simulink model "TB23_R2_SALS_Link"  (R2025a)
settings: Solver=FixedStepDiscrete  StartTime=0  StopTime=TB.t_end  FixedStep=TB.dt  RelTol=1e-3
InitFcn:
  | % 모델과 같은 폴더의 초기화 스크립트를 실행해 P(설계 파라미터)와 TB(시험 조건)를 만든다.
  | run(fullfile(fileparts(get_param(bdroot, 'FileName')), 'TB23_init.m'));
values from neighbouring files (symbols this model uses):
  TB = struct()    [TB23_init.m]    (also in run_TB23.m = evalin('base', 'TB'))
libraries: fl_lib x71, nesl_utility x31
(part 3 of 3)

== matlab function TB23_R2_SALS_Link/Gate_StageB/StageB_Gate ==
  data: t input; g output; uc input; ilink input; prm input; init input; eps input; aux output
function [g, aux] = prism_gate_stageB_f(t, uc, ilink, prm, init, eps)
%#codegen
%PRISM_GATE_STAGEB_F  Stage B 게이트 생성기 + DAB 고장 모드 변조(EPS) + 직류 편류 없는 지령 전이(TB12).
%
%  ctrl/prism_gate_stageB_e.m(TB10·TB11)과 같고, EPS 지령이 바뀔 때의 전이만 다르다(TB11에서 지령표 칸 전환으로
%  (D1, φ)가 한 번에 0.1·0.23 rad 바뀐 주기에 누설 전류에 직류 편류가 생겨 첨두가 88.5 A까지 올랐다).
%    1) 레그 2 지연(D1)이 바뀌면 그 뒤 첫 레그 2 에지는 이전·새 값의 중간(반 이동), 다음 에지부터 새 값을 쓴다.
%       구형파 레그 하나의 에지가 Δ 옮겨질 때 첫 에지를 Δ/2만 옮기면 그 레그가 만드는 인덕터 전류에 직류 편류가 남지 않는다
%       (SPS 위상의 전이 반주기 평균과 같은 원리를 레그마다 적용). 이전 판(e)은 D1을 한 주기 동안 그대로 잡았다.
%    2) EPS 위상은 반주기마다 SPH = 0.01 rad, D1은 에지마다 SD1 = 0.005까지만 옮긴다(지령표의 큰 칸 전환을 수 주기에 나눔).
%       EPS가 켜질 때는 지금 쓰던 SPS 위상에서 출발한다. 정상 붕괴 중의 지령 변화(주기당 D1 약 0.0006)보다 훨씬 크므로
%       평소 동작에는 영향이 없다.
%  EPS가 꺼져 있으면(eps(1) = 0) prism_gate_stageB.m·prism_gate_stageB_e.m과 같은 게이트를 낸다.
%  아래는 이전 판 설명:
%PRISM_GATE_STAGEB_E(이전 판)  Stage B 게이트 생성기 + DAB 고장 모드 변조(EPS, TB10). eps(1) = 0이면 ctrl/prism_gate_stageB.m과 같다.
%
%  EPS(1차 내부 위상천이): SPS 생성기가 정한 1차 에지(가상 에지)에서 레그 1(P1·P2)은 그대로 바꾸고, 레그 2(P3·P4)는
%  D1·T/2 늦게 바꾼다. 1차 전압은 −V → 0(레그 1만 바뀜) → +V(레그 2도 바뀜)가 되어 반주기마다 (1 − D1)·T/2 폭의 펄스가 된다.
%  D1은 상향 가상 에지에서 잡아 그 주기의 하향 에지까지 그대로 쓴다(양·음 펄스 폭이 같아 1차 직류 편류가 생기지 않는다).
%  위상은 eps(2)를 SPS 위상 지령 대신 쓰므로, 위상 변화의 직류 편류 방지(전이 반주기 평균)는 SPS와 같이 적용된다.
%  위상 기준: 2차 상향 에지 − 가상 에지 = φ, 1차 펄스 시작 = 가상 에지 + D1·T/2(검증 코드 dab_modulation.eps_params와 같은 정의).
%
%  추가 입력  eps  [EPS 켬(1/0); 위상 φ [rad]; 내부 위상비 D1(0–0.95)]  (ctrl/prism_dab_eps_map.m)
%
%  아래는 SPS 생성기 설명(그대로):
%PRISM_GATE_STAGEB  Stage B 게이트 생성기(적분 간격 dt = 5 ns마다 실행).
%
%  H-브리지 : 유니폴라 PWM. 삼각 반송파 c(t)는 제어주기 시작(표본 시점)에서 +1, 반주기에서 −1.
%             레그 A 상측 목표 = (m > c), 레그 B 상측 목표 = (−m > c). 목표가 바뀌면 두 소자를 데드타임 동안
%             끄고(출력용량 충방전·다이오드 도통은 회로가 정함) 새 소자를 켠다.
%  DAB      : 50 % 구형파 두 풀브리지, 단일 위상천이. 에지는 반송파 반주기 중심 c_j에 대칭(1차 c_j − δ/2,
%             2차 c_j + δ/2, δ = φ·T/2π)으로 놓고, 지령은 도착 후 첫 반주기 중심에서 반영한다.
%             전이 반주기의 위상차를 이전·새 위상의 평균으로 두는 갱신(A ← −A + 2Δ, Δ = (A + δ_new)/2)으로
%             위상이 바뀔 때 변압기 직류 편류가 생기지 않게 한다(검증 코드와 같은 알고리즘).
%             에지 시각은 dt 격자에 반올림하고, 실제 실행 시각으로 다음 반주기의 A를 계산한다.
%  링크전류 : DAB 2차 브리지가 링크로 보내는 직류전류를 제어주기마다 평균해 다음 표본에 넘긴다.
%
%  입력  t      시뮬레이션 시각(Digital Clock, dt 간격)
%        uc     [PWM 비교값; DAB 유효 위상 rad]  (제어기 출력, 전달지연 뒤)
%        ilink  DAB 2차 브리지 → 링크 직류전류 [A](순시)
%        prm    [dt Np td_h(간격 수) td_d(간격 수) T]
%        init   [PWM 비교값 초기값, 위상 초기값, 링크전류 초기값]
%  출력  g      [A상측 A하측 B상측 B하측 | P1 P2 P3 P4 | S1 S2 S3 S4]  (1 = 켬)
%               DAB 브리지: 상태 +1 → 1·4번 켬, −1 → 2·3번 켬(1·2번이 레그 1, 3·4번이 레그 2, 홀수 = 상측)
%        aux    [링크전류 주기 평균; 그 주기 두 반주기 중심의 위상 φ_c0, φ_c1; 반송파; 1차 상태; 2차 상태]

persistent started kA kB tgtA tgtB A ph_tgt p_t s_t p_h s_h p_j s_j p_state s_state p_te s_te ...
           acc il_avg phc0 phc1 lat0 lat1 D1c l2_t l2_tgt l2_hi l2_te l2_pend D1p ph_e e_on
dt = prm(1); Np = prm(2); ndh = prm(3); ndd = prm(4); T = prm(5);
Nh = round(Np/2);
k  = round(t/dt);                     % 적분 간격 번호(0부터)
t0 = k*dt;

if isempty(started)
    started = 1;
    m0 = init(1); ph0 = init(2);
    c0 = 1;                            % k = 0의 반송파
    tgtA = double(m0 > c0); tgtB = double(-m0 > c0);
    kA = -1e9; kB = -1e9;              % 데드타임 없이 시작
    ph_tgt = ph0;
    d0 = ph0/(2*pi)*T;
    A = d0;
    p_t = [1e30 1e30]; s_t = [1e30 1e30]; p_h = [0 0]; s_h = [0 0];
    p_te = -1; s_te = -1;
    if d0 > 0
        p_j = 1; p_h(1) = -d0/2; p_state = 1;  s_j = 0; s_state = -1;
    elseif d0 < 0
        s_j = 1; s_h(1) = d0/2;  s_state = 1;  p_j = 0; p_state = -1;
    else
        p_j = 0; s_j = 0; p_state = -1; s_state = -1;
    end
    acc = 0; il_avg = init(3); phc0 = ph0; phc1 = ph0; lat0 = ph0; lat1 = ph0;
    D1c = 0; D1p = 0; ph_e = 0; e_on = 0; l2_t = 1e30; l2_tgt = double(p_state < 0); l2_hi = l2_tgt; l2_te = -1; l2_pend = 0;
end

m = uc(1);
SPH = 0.01;                           % EPS 위상 변화율 상한 [rad/반주기]
SD1 = 0.005;                          % EPS D1 변화율 상한 [/반주기]
if eps(1) > 0.5
    if ~e_on, ph_e = ph_tgt; e_on = 1; end           % 켜질 때 지금 쓰는 SPS 위상에서 출발
    if mod(k, Nh) == 0                               % 반주기 중심에서만 위상 지령을 한 단계 옮긴다
        dphi = mod(eps(2) - ph_e + pi, 2*pi) - pi;
        ph_e = ph_e + min(max(dphi, -SPH), SPH);
    end
    ph_tgt = ph_e;
else
    e_on = 0;
    ph_tgt = uc(2);
end

% ---------------- H-브리지 유니폴라 PWM -------------------------------------------------
kin = mod(k, Np);
c = 4*abs(kin/Np - 0.5) - 1;
nA = double(m > c); nB = double(-m > c);
if nA ~= tgtA, tgtA = nA; kA = k; end
if nB ~= tgtB, tgtB = nB; kB = k; end
okA = (k - kA) >= ndh; okB = (k - kB) >= ndh;
gA_hi = double(okA && tgtA == 1); gA_lo = double(okA && tgtA == 0);
gB_hi = double(okB && tgtB == 1); gB_lo = double(okB && tgtB == 0);

% ---------------- DAB 위상 갱신(반주기 중심) --------------------------------------------
if mod(k, Nh) == 0
    j = k/Nh; cj = t0;
    if j >= 1
        jm = mod(j - 1, 2) + 1;
        A = -A + 2*(s_h(jm) - p_h(jm));
    end
    dtg = ph_tgt/(2*pi)*T;
    D = 0.5*(A + dtg);
    jj = mod(j, 2) + 1;
    p_done = p_j > j; s_done = s_j > j;
    if p_done && ~s_done
        s_t(jj) = max(cj, p_h(jj) + D);
    elseif s_done && ~p_done
        p_t(jj) = max(cj, s_h(jj) - D);
    elseif ~p_done && ~s_done
        if D >= 0
            p_t(jj) = cj; s_t(jj) = cj + D;
        else
            s_t(jj) = cj; p_t(jj) = cj - D;
        end
    end
    if p_done, tpj = p_h(jj); else, tpj = p_t(jj); end
    if s_done, tsj = s_h(jj); else, tsj = s_t(jj); end
    D1 = 0.5*(-A + 2*(tsj - tpj) + dtg);
    cn = (j + 1)*Nh*dt;
    p_t(3 - jj) = cn - D1/2; s_t(3 - jj) = cn + D1/2;
    if mod(j, 2) == 0, phc0 = ph_tgt; else, phc1 = ph_tgt; end
end
% ---------------- DAB 에지 실행(가장 가까운 간격에 반올림) ------------------------------
sp = mod(p_j, 2) + 1;
if p_t(sp) < t0 + 0.5*dt
    if mod(p_j, 2) == 0, p_state = 1; else, p_state = -1; end
    if eps(1) > 0.5, D1n = min(max(eps(3), 0), 0.95); else, D1n = 0; end
    D1n = D1p + min(max(D1n - D1p, -SD1), SD1);      % 에지마다 D1 변화율 제한
    if abs(D1n - D1p) > 1e-9
        D1c = 0.5*(D1p + D1n);        % 레그 2 지연이 바뀌면 첫 에지는 중간값(반 이동), 다음 에지부터 새 값: 직류 편류 없음
        D1p = D1n;
    else
        D1c = D1n;
    end
    p_te = t0; p_h(sp) = t0; p_t(sp) = 1e30; p_j = p_j + 1;
    if l2_pend > 0.5                   % (위상 전이로 반주기가 짧아진 경우) 남은 레그 2 전환을 먼저 끝낸다
        l2_hi = l2_tgt; l2_te = t0; l2_pend = 0;
    end
    l2_tgt = double(p_state < 0); l2_t = t0 + D1c*T/2; l2_pend = 1;   % 레그 2: −1 상태에서 상측(P3) 켬
end
if l2_pend > 0.5 && l2_t < t0 + 0.5*dt
    l2_hi = l2_tgt; l2_te = t0; l2_pend = 0;
end
ss = mod(s_j, 2) + 1;
if s_t(ss) < t0 + 0.5*dt
    if mod(s_j, 2) == 0, s_state = 1; else, s_state = -1; end
    s_te = t0; s_h(ss) = t0; s_t(ss) = 1e30; s_j = s_j + 1;
end
p_ok = (t0 - p_te) >= ndd*dt - 0.5*dt;
s_ok = (t0 - s_te) >= ndd*dt - 0.5*dt;
gP = [0 0 0 0]; gS = [0 0 0 0];
if p_ok                                % 레그 1(P1 상측, P2 하측)
    if p_state > 0, gP(1:2) = [1 0]; else, gP(1:2) = [0 1]; end
end
if (t0 - l2_te) >= ndd*dt - 0.5*dt     % 레그 2(P3 상측, P4 하측), 자기 전환 뒤 데드타임
    if l2_hi > 0.5, gP(3:4) = [1 0]; else, gP(3:4) = [0 1]; end
end
if s_ok
    if s_state > 0, gS = [1 0 0 1]; else, gS = [0 1 1 0]; end
end

% ---------------- 링크전류 주기 평균(표본 직전 간격에서 확정) -------------------------
acc = acc + ilink;
if kin == Np - 1
    il_avg = acc/Np; acc = 0;
    lat0 = phc0; lat1 = phc1;
end

g = [gA_hi gA_lo gB_hi gB_lo gP gS]';
aux = [il_avg; lat0; lat1; c; p_state; s_state];
end

== matlab function TB23_R2_SALS_Link/Gate_StageB/R2_Gate_Protect ==
  data: t input; gb output; g input; sup input; meas input; prm input; fl output
function [gb, fl] = prism_r2_gate_b(t, g, sup, meas, prm)
%#codegen
%PRISM_R2_GATE_B  R2 보호 상태기계의 게이트 재정의(TB09, 적분 간격마다 실행): 하드웨어 비교기, 고장 주입, 모드별 게이트.
%
%  입력  g     게이트 생성기 출력 [A상측 A하측 B상측 B하측 | P1–P4 | S1–S4] (ctrl/prism_gate_stageB.m)
%        sup   상태기계 지령 [브리지 모드(0 제어 PWM, 1 영벡터, 2 차단, 3 조향 PWM); DAB 모드(0 제어기, 1 보조, 2 정지);
%              바이패스 주 스위치; 제동 저항 게이트; 상태 번호]
%        meas  [i_p i_h v_link v_s v_bus]
%        prm   [dt T_HW I_HW VL_HW VS_HW 상한 고장종류(0 없음, 1 H-브리지 개방, 2 DAB 정지) 고장시각 T_GDF (두 번째 고장 시각)]
%              (TB23) 10번째 값이 있으면 그 시각에 비교기 차단 래치를 강제로 켠다(DAB 고장 강등 중 H-브리지 차단 → 이중 고장)
%  출력  gb    [H-브리지 4 | DAB 8 | 바이패스 주 스위치 | 제동 저항]
%        fl    [게이트 구동기 고장 신호(H-브리지 개방, T_GDF 뒤); 하드웨어 비교기 차단 래치]
%  하드웨어 비교기는 H-브리지가 동작하는 동안(차단·고장 전) 연속 감시한다: |i_p|·|i_h| > I_HW, v_link > VL_HW,
%  |v_s| > VS_HW, 그리고 정상 조정 상태(1–5)에서 v_bus > 부품 등급 상한. 조건이 T_HW 동안 이어지면 브리지를 끄고 래치한다.

persistent since trip
if isempty(trip), since = -1; trip = 0; end
T_HW = prm(2); I_HW = prm(3); VL_HW = prm(4); VS_HW = prm(5); upper = prm(6);
ftype = prm(7); t_f = prm(8); T_GDF = prm(9);
bmode = round(sup(1)); dmode = round(sup(2)); st = round(sup(5));
hb_fault = ftype == 1 && t >= t_f;
dab_fault = ftype == 2 && t >= t_f;
ip = meas(1); ih = meas(2); vl = meas(3); vs = meas(4); vb = meas(5);
if trip < 0.5 && ~hb_fault && bmode ~= 2
    normal = st >= 1 && st <= 5;
    cond = abs(ip) > I_HW || abs(ih) > I_HW || vl > VL_HW || abs(vs) > VS_HW || (normal && vb > upper);
    if cond
        if since < 0, since = t; end
        if t - since >= T_HW - 1e-15, trip = 1; end
    else
        since = -1;
    end
end
if numel(prm) >= 10 && t >= prm(10)
    trip = 1;                                     % (TB23) 두 번째 고장 주입
end
gb = [g(:); 0; 0];
if trip > 0.5 || hb_fault || bmode == 2
    gb(1:4) = 0;
elseif bmode == 1
    gb(1:4) = [0; 1; 0; 1];                       % 영벡터: H-브리지 하측 두 소자
end
if dab_fault || dmode == 2
    gb(5:12) = 0;
end
gb(13) = double(sup(3) > 0.5);
gb(14) = double(sup(4) > 0.5);
fl = [double(hb_fault && t >= t_f + T_GDF); trip];
end

== matlab function TB23_R2_SALS_Link/Gate_StageB/DAB_EPS_Map ==
  data: sup input; eps output; meas input; prm input; tD input; tP input; tK input
function eps = prism_dab_eps_map(sup, meas, prm, tD, tP, tK)
%#codegen
%PRISM_DAB_EPS_MAP  H-브리지 고장 강등 중 DAB 고장 모드 변조(EPS) 지령(TB10, 검증 코드 E20과 같은 표).
%
%  강등 상태(9 유지, 10 링크 붕괴, 11 소프트 투입)에서 DAB 모드가 보조 지령(1)이면, 상태기계의 보조 링크전류 지령을
%  1차 내부 위상천이(EPS) 지령 [등가 위상 φ; 내부 위상비 D1]로 바꾼다. 게이트 생성기(ctrl/prism_gate_stageB_e.m)는
%  1차 두 레그 가운데 레그 2를 D1·T/2만큼 늦춰 1차 전압에 영구간을 넣고, 2차는 φ만큼 위상을 둔 구형파로 둔다.
%
%  정규화(2차 환산): V1' = v_bus/n, ωL' = 2π f_s L_dab/n², I_b = V1'/ωL', r = v_link/V1', j = 지령/I_b.
%  표(검증 코드 dab_modulation.py가 만든 것을 TB10_init.m이 읽음): r(행) × j(열, −0.78–0, 링크 → 1차만)마다
%    tD 1차 펄스 폭 d [rad](D1 = 1 − d/π), tP 등가 위상 φ [rad], tK 정규화 첨두.
%  첨두 상한: 같은 r에서 tK ≤ pk_max/I_b인 가장 큰 |j|까지만 지령한다(나머지 링크전력은 제동 저항이 받음).
%  링크를 채우는 지령(j > 0)은 내지 않는다(강등 중 링크는 다이오드 정류 전류로 채워진다).
%
%  입력  sup   상태기계 지령 12개(5 DAB 모드, 6 보조 링크전류 지령, 11 상태)
%        meas  [v_bus v_link]
%        prm   [켬 n L_dab f_s pk_max r0 dr j0 dj]
%  출력  eps   [EPS 켬; φ; D1]

on = prm(1) > 0.5 && round(sup(5)) == 1 && round(sup(11)) >= 9 && round(sup(11)) <= 11;
eps = [0; 0; 0];
if ~on
    return
end
n = prm(2); Ld = prm(3); fs = prm(4); pkmax = prm(5);
r0 = prm(6); dr = prm(7); j0 = prm(8); dj = prm(9);
[nr, nj] = size(tD);
v1 = max(meas(1), 1)/n;
Ib = v1/(2*pi*fs*Ld/(n*n));
r = min(max(meas(2)/v1, r0), r0 + (nr - 1)*dr);
ir = min(floor((r - r0)/dr) + 1, nr - 1); fr = (r - r0)/dr - (ir - 1);
% 첨두 상한을 지키는 최대 |j|(j = 0 열에서 음의 방향으로)
tgt = pkmax/Ib;
jl = 0;
for k = nj:-1:1
    pk = (1 - fr)*tK(ir, k) + fr*tK(ir + 1, k);
    if pk > tgt
        break
    end
    jl = -(j0 + (k - 1)*dj);
end
jn = min(max(sup(6)/Ib, -jl), 0);
jn = max(jn, j0);
ij = min(floor((jn - j0)/dj) + 1, nj - 1); fj = (jn - j0)/dj - (ij - 1);
d  = (1 - fr)*(1 - fj)*tD(ir, ij) + (1 - fr)*fj*tD(ir, ij + 1) + fr*(1 - fj)*tD(ir + 1, ij) + fr*fj*tD(ir + 1, ij + 1);
ph = (1 - fr)*(1 - fj)*tP(ir, ij) + (1 - fr)*fj*tP(ir, ij + 1) + fr*(1 - fj)*tP(ir + 1, ij) + fr*fj*tP(ir + 1, ij + 1);
D1 = min(max(1 - d/pi, 0), 0.95);
eps = [1; ph; D1];
end
